simulink model "sparrow_albatros_spec_withgpio"  (R2021a)
settings: Solver=VariableStepDiscrete  StartTime=0.0  StopTime=100  RelTol=1e-3
undefined symbols (not defined in the file): pfb_coeff_gen_calc
libraries: xbsIndex_r4 x5582, casper_library_misc x33, casper_library_delays x28, xps_library x10, simulink x8, xbsReplacements_r4 x2
(part 8 of 80)

== system sparrow_albatros_spec_withgpio/reorder ==
  sync : Inport
  en : Inport  Port=2
  din0 : Inport  Port=3
  delay_din0 : xbsIndex_r4/Delay  rst=off  infoeditControl=Selection of Reset will increase slice count due to use of real FFs and instead of SRLs  en=off  latency=3  reg_retiming=on  dbl_ovrd=off  block_type=delay
  delay_din_bram0 : casper_library_delays/delay_bram_en_plus  DelayLen=length(map)  bram_latency=bram_latency+fanout_latency
      settings: SourceProductName=CASPER DSP Blockset
  delay_valid : xbsIndex_r4/Delay  rst=off  infoeditControl=Selection of Reset will increase slice count due to use of real FFs and instead of SRLs  en=off  latency=3  reg_retiming=on  dbl_ovrd=off  block_type=delay
  delay_we0 : xbsIndex_r4/Delay  rst=off  infoeditControl=Selection of Reset will increase slice count due to use of real FFs and instead of SRLs  en=off  latency=3  reg_retiming=on  dbl_ovrd=off  block_type=delay
  delay_we1 : xbsIndex_r4/Delay  rst=off  infoeditControl=Selection of Reset will increase slice count due to use of real FFs and instead of SRLs  en=off  latency=3  reg_retiming=on  dbl_ovrd=off  block_type=delay
  delay_we2 : xbsIndex_r4/Delay  rst=off  infoeditControl=Selection of Reset will increase slice count due to use of real FFs and instead of SRLs  en=off  latency=3  reg_retiming=on  dbl_ovrd=off  block_type=delay
  or : xbsIndex_r4/Logical  logical_function=OR  inputs=2  en=off  latency=0  precision=Full  arith_type=Unsigned  n_bits=16  bin_pt=0  align_bp=on  dbl_ovrd=off  block_type=logical
  post_sync_delay : xbsIndex_r4/Delay  rst=off  infoeditControl=Selection of Reset will increase slice count due to use of real FFs and instead of SRLs  en=off  latency=3  reg_retiming=on  dbl_ovrd=off  block_type=delay
  pre_sync_delay : xbsIndex_r4/Delay  rst=off  infoeditControl=Selection of Reset will increase slice count due to use of real FFs and instead of SRLs  en=off  latency=3  reg_retiming=on  dbl_ovrd=off  block_type=delay
  sync_delay_en : casper_library_delays/sync_delay_en  DelayLen=2048
      settings: SourceProductName=CASPER DSP Blockset
  we_expand : Subsystem  AncestorBlock=casper_library_flow_control/bus_expand  mask(bus_expand){mode=divisions of equal size, outputNum=1, outputWidth=1, outputBinaryPt=0, outputArithmeticType=2, show_format=off, outputToWorkspace=off, variablePrefix=out, outputToModelAsWell=on}
      mask prompts: outputNum "Number of outputs:"; outputWidth "Output width:"; outputBinaryPt "Output binary point position:"; outputArithmeticType "Output arithmetic type (ufix=0, fix=1, bool=2):"; show_format "Print format string?"; outputToWorkspace "Output to workspace?"; variablePrefix "Variable name prefix:"; outputToModelAsWell "Output to model as well?"
      mask help:
      | Expands a 'bus' made using a bus_create or Xilinx
      | concat block.
      | The input will be divided into the specified number
      | of outputs with the specified arithmetic types.
      | Divisions are made from most significant bit.
      mask init: same as sparrow_albatros_spec_withgpio/bus_expand
      settings: AttributesFormatString=1 outputs
      mask TypeOptions mode: divisions of equal size | divisions of arbitrary size
      mask Callback mode: %bus_expand_callback();
      mask Callback outputWidth: %bus_expand_callback();
      mask Callback outputToWorkspace: %bus_expand_callback();
  we_replicate : Subsystem  AncestorBlock=casper_library_bus/bus_replicate  mask(bus_replicate){replication=1, csp_latency=0, misc=off, implementation=core}
      mask prompts: replication "replication factor"; csp_latency "latency"; misc "misc support"; implementation "delay implementation"
      mask help: Output bus formed by replicating input bus a number of times
      mask init:
      | bus_replicate_init(gcb, ...
      |     'replication', replication, ...
      |     'csp_latency', csp_latency, ...
      |     'implementation', implementation, ...
      |     'misc', misc);
      mask TypeOptions implementation: core | behavioral
  sync_out : Outport
  valid : Outport  Port=2
  dout0 : Outport  Port=3
  wires:
  en/1 -> delay_we0/1, delay_we1/1, delay_we2/1
  delay_we1/1 -> delay_valid/1
  delay_valid/1 -> valid/1
  delay_we2/1 -> we_replicate/1(in)
  we_replicate/1(out) -> we_expand/1(bus_in)
  sync/1 -> pre_sync_delay/1
  delay_we0/1 -> or/2
  pre_sync_delay/1 -> or/1, sync_delay_en/1
  or/1 -> sync_delay_en/2
  sync_delay_en/1 -> post_sync_delay/1
  post_sync_delay/1 -> sync_out/1
  din0/1 -> delay_din0/1
  delay_din0/1 -> delay_din_bram0/1
  delay_din_bram0/1 -> dout0/1
  we_expand/1(msb_lsb_out1) -> delay_din_bram0/2

== system sparrow_albatros_spec_withgpio/sel ==
  sim_1 : Inport
  convert1_1 : DataTypeConversion  OutDataTypeStr=fixdt('ufix1_En0')  LockScale=on
  convert2_1 : DataTypeConversion  OutDataTypeStr=fixdt('ufix1_En0')  ConvertRealWorld=Stored Integer (SI)  LockScale=on
  gain_1 : Gain  OutDataTypeStr=fixdt('ufix32_En0')
  io_delay : xbsIndex_r4/Delay  rst=off  infoeditControl=Selection of Reset will increase slice count due to use of real FFs and instead of SRLs  en=off  latency=0  reg_retiming=on  dbl_ovrd=off  block_type=delay
  slice_reg : xbsIndex_r4/Slice  nbits=1  boolean_output=on  mode=Lower Bit Location + Width  bit1=0  base1=MSB of Input  bit0=0  base0=LSB of Input  dbl_ovrd=off  block_type=slice
  sparrow_albatros_spec_withgpio_sel_user_data_out : xbsIndex_r4/Gateway In  gui_display_data_type=Fixed-point  arith_type=Unsigned  n_bits=32  bin_pt=0  preci_type=Single  exp_width=8  frac_width=24  rows=1  columns=1  quantization="Round  (unbiased: +/- Inf)"  overflow=Saturate  period=1  UseAsADC=off  ADCChannel='1'  interface=None  automatic_assignment=on  address_offset=hex2dec('00')  intf_name=''  intf_description=''  default_value=0  timing_constraint=None  locs_specified=off  LOCs={}  io_standard={}  inherit_from_input=off  hdl_port=on  dbl_ovrd=off  block_type=gatewayin
  in_reg : Outport  VectorParamsAs1DForOutWhenUnconnected=off
  wires:
  sparrow_albatros_spec_withgpio_sel_user_data_out/1 -> io_delay/1
  sim_1/1 -> convert1_1/1
  convert1_1/1 -> convert2_1/1
  convert2_1/1 -> gain_1/1
  gain_1/1 -> sparrow_albatros_spec_withgpio_sel_user_data_out/1
  io_delay/1 -> slice_reg/1
  slice_reg/1 -> in_reg/1

== system sparrow_albatros_spec_withgpio/sim_pulse_gen ==
  Compare To Constant : simulink/Logic and Bit Operations/Compare To Constant  relop===  const=delay  OutDataTypeStr=boolean
  Counter Limited : simulink/Sources/Counter Limited  uplimit=delay+1  tsamp=-1
  Logical Operator : Logic  AllPortsSameDT=off  OutDataTypeStr=boolean
  Logical Operator1 : Logic  AllPortsSameDT=off  OutDataTypeStr=boolean
  Logical Operator2 : Logic  Operator=NOT  AllPortsSameDT=off  OutDataTypeStr=boolean
  Memory : Memory  InitialCondition=1
  Out1 : Outport
  wires:
  Logical Operator1/1 -> Memory/1
  Logical Operator/1 -> Out1/1, Logical Operator2/1
  Counter Limited/1 -> Compare To Constant/1
  Compare To Constant/1 -> Logical Operator/1
  Logical Operator2/1 -> Logical Operator1/2
  Memory/1 -> Logical Operator1/1, Logical Operator/2

== system sparrow_albatros_spec_withgpio/sim_pulse_gen1 ==
  Compare To Constant : simulink/Logic and Bit Operations/Compare To Constant  relop===  const=delay  OutDataTypeStr=boolean
  Counter Limited : simulink/Sources/Counter Limited  uplimit=delay+1  tsamp=-1
  Logical Operator : Logic  AllPortsSameDT=off  OutDataTypeStr=boolean
  Logical Operator1 : Logic  AllPortsSameDT=off  OutDataTypeStr=boolean
  Logical Operator2 : Logic  Operator=NOT  AllPortsSameDT=off  OutDataTypeStr=boolean
  Memory : Memory  InitialCondition=1
  Out1 : Outport
  wires:
  Memory/1 -> Logical Operator/2, Logical Operator1/1
  Logical Operator2/1 -> Logical Operator1/2
  Compare To Constant/1 -> Logical Operator/1
  Counter Limited/1 -> Compare To Constant/1
  Logical Operator/1 -> Logical Operator2/1, Out1/1
  Logical Operator1/1 -> Memory/1

== system sparrow_albatros_spec_withgpio/sim_pulse_gen2 ==
  Compare To Constant : simulink/Logic and Bit Operations/Compare To Constant  relop===  const=delay  OutDataTypeStr=boolean
  Counter Limited : simulink/Sources/Counter Limited  uplimit=delay+1  tsamp=-1
  Logical Operator : Logic  AllPortsSameDT=off  OutDataTypeStr=boolean
  Logical Operator1 : Logic  AllPortsSameDT=off  OutDataTypeStr=boolean
  Logical Operator2 : Logic  Operator=NOT  AllPortsSameDT=off  OutDataTypeStr=boolean
  Memory : Memory  InitialCondition=1
  Out1 : Outport
  wires:
  Logical Operator1/1 -> Memory/1
  Logical Operator/1 -> Out1/1, Logical Operator2/1
  Counter Limited/1 -> Compare To Constant/1
  Compare To Constant/1 -> Logical Operator/1
  Logical Operator2/1 -> Logical Operator1/2
  Memory/1 -> Logical Operator1/1, Logical Operator/2

== system sparrow_albatros_spec_withgpio/simple_bram_vacc2 ==
  new_acc : Inport
  din : Inport  Port=2
  Adder : xbsIndex_r4/AddSub  mode=Addition  use_carryin=off  use_carryout=off  en=off  latency=2  precision=User Defined  arith_type=Unsigned  n_bits=n_bits  bin_pt=bin_pt  quantization=Truncate  overflow=Wrap  use_behavioral_HDL=on  hw_selection=Fabric  pipelined=off  use_rpm=on  dbl_ovrd=off  block_type=addsub
      settings: xl_area=[0, 0, 0, 0, 0, 0, 0]  block_version=10.1.3
  Constant : xbsIndex_r4/Constant  const=0  gui_display_data_type=Fixed-point  arith_type=Unsigned  n_bits=n_bits  bin_pt=bin_pt  preci_type=Single  exp_width=8  frac_width=24  explicit_period=on  period=1  equ=P=C  opselect=C  inp2=PCIN>>17  opr=+  inp1=P  carry=CIN  dbl_ovrd=off  block_type=constant
  Mux : xbsIndex_r4/Mux  inputs=2  en=off  latency=0  precision=Full  arith_type="Signed  (2's comp)"  n_bits=8  bin_pt=2  quantization=Truncate  overflow=Wrap  dbl_ovrd=off  block_type=mux
      settings: xl_area=[0, 0, 0, 0, 0, 0, 0]
  delay_bram : Subsystem  mask(delay_bram){DelayLen=vec_len - 2, bram_latency=2}
      mask prompts: DelayLen "Delay By:"; bram_latency "BRAM Latency"
      mask help: A delay block that uses BRAM for its storage.
      mask init:
      | if (DelayLen <= bram_latency)
      | 	error('delay value must be greater than BRAM Latency');
      | end
      | BitWidth = max(ceil(log2(DelayLen)), 2);
      mask Help: eval('xlWeb(''http://casper.berkeley.edu/wiki/Delay_bram'')')
  pulse_ext : Subsystem  mask(pulse_ext){pulse_len=vec_len}
      mask prompts: pulse_len "Length of Pulse"
      mask help:
      | Extends a boolean signal to be high for the specified number of clocks after
      | the last high input.
      mask init:
      | bits = ceil(log2(pulse_len+1));
      mask Help: eval('xlWeb(''http://casper.berkeley.edu/wiki/Pulse_ext'')')
  dout : Outport  VectorParamsAs1DForOutWhenUnconnected=off
  valid : Outport  Port=2  VectorParamsAs1DForOutWhenUnconnected=off
  wires:
  Adder/1 -> delay_bram/1(In1)
  delay_bram/1(Out1) -> dout/1, Mux/2
  new_acc/1 -> pulse_ext/1(in)
  din/1 -> Adder/1
  pulse_ext/1(out) -> valid/1, Mux/1
  Mux/1 -> Adder/2
  Constant/1 -> Mux/3

== system sparrow_albatros_spec_withgpio/simple_bram_vacc3 ==
  new_acc : Inport
  din : Inport  Port=2
  Adder : xbsIndex_r4/AddSub  mode=Addition  use_carryin=off  use_carryout=off  en=off  latency=2  precision=User Defined  arith_type=Unsigned  n_bits=n_bits  bin_pt=bin_pt  quantization=Truncate  overflow=Wrap  use_behavioral_HDL=on  hw_selection=Fabric  pipelined=off  use_rpm=on  dbl_ovrd=off  block_type=addsub
      settings: xl_area=[0, 0, 0, 0, 0, 0, 0]  block_version=10.1.3
  Constant : xbsIndex_r4/Constant  const=0  gui_display_data_type=Fixed-point  arith_type=Unsigned  n_bits=n_bits  bin_pt=bin_pt  preci_type=Single  exp_width=8  frac_width=24  explicit_period=on  period=1  equ=P=C  opselect=C  inp2=PCIN>>17  opr=+  inp1=P  carry=CIN  dbl_ovrd=off  block_type=constant
  Mux : xbsIndex_r4/Mux  inputs=2  en=off  latency=0  precision=Full  arith_type="Signed  (2's comp)"  n_bits=8  bin_pt=2  quantization=Truncate  overflow=Wrap  dbl_ovrd=off  block_type=mux
      settings: xl_area=[0, 0, 0, 0, 0, 0, 0]
  delay_bram : Subsystem  mask(delay_bram){DelayLen=vec_len - 2, bram_latency=2}
      mask prompts: DelayLen "Delay By:"; bram_latency "BRAM Latency"
      mask help: A delay block that uses BRAM for its storage.
      mask init:
      | if (DelayLen <= bram_latency)
      | 	error('delay value must be greater than BRAM Latency');
      | end
      | BitWidth = max(ceil(log2(DelayLen)), 2);
      mask Help: eval('xlWeb(''http://casper.berkeley.edu/wiki/Delay_bram'')')
  pulse_ext : Subsystem  mask(pulse_ext){pulse_len=vec_len}
      mask prompts: pulse_len "Length of Pulse"
      mask help:
      | Extends a boolean signal to be high for the specified number of clocks after
      | the last high input.
      mask init:
      | bits = ceil(log2(pulse_len+1));
      mask Help: eval('xlWeb(''http://casper.berkeley.edu/wiki/Pulse_ext'')')
  dout : Outport  VectorParamsAs1DForOutWhenUnconnected=off
  valid : Outport  Port=2  VectorParamsAs1DForOutWhenUnconnected=off
  wires:
  Constant/1 -> Mux/3
  Mux/1 -> Adder/2
  pulse_ext/1(out) -> Mux/1, valid/1
  din/1 -> Adder/1
  new_acc/1 -> pulse_ext/1(in)
  delay_bram/1(Out1) -> Mux/2, dout/1
  Adder/1 -> delay_bram/1(In1)

== system sparrow_albatros_spec_withgpio/simple_bram_vacc4 ==
  new_acc : Inport
  din : Inport  Port=2
  Adder : xbsIndex_r4/AddSub  mode=Addition  use_carryin=off  use_carryout=off  en=off  latency=2  precision=User Defined  arith_type="Signed  (2's comp)"  n_bits=n_bits  bin_pt=bin_pt  quantization=Truncate  overflow=Wrap  use_behavioral_HDL=on  hw_selection=Fabric  pipelined=off  use_rpm=on  dbl_ovrd=off  block_type=addsub
      settings: xl_area=[0, 0, 0, 0, 0, 0, 0]  block_version=10.1.3
  Constant : xbsIndex_r4/Constant  const=0  gui_display_data_type=Fixed-point  arith_type=Signed (2's comp)  n_bits=n_bits  bin_pt=bin_pt  preci_type=Single  exp_width=8  frac_width=24  explicit_period=on  period=1  equ=P=C  opselect=C  inp2=PCIN>>17  opr=+  inp1=P  carry=CIN  dbl_ovrd=off  block_type=constant
  Mux : xbsIndex_r4/Mux  inputs=2  en=off  latency=0  precision=Full  arith_type="Signed  (2's comp)"  n_bits=8  bin_pt=2  quantization=Truncate  overflow=Wrap  dbl_ovrd=off  block_type=mux
      settings: xl_area=[0, 0, 0, 0, 0, 0, 0]
  delay_bram : Subsystem  mask(delay_bram){DelayLen=vec_len - 2, bram_latency=2}
      mask prompts: DelayLen "Delay By:"; bram_latency "BRAM Latency"
      mask help: A delay block that uses BRAM for its storage.
      mask init:
      | if (DelayLen <= bram_latency)
      | 	error('delay value must be greater than BRAM Latency');
      | end
      | BitWidth = max(ceil(log2(DelayLen)), 2);
      mask Help: eval('xlWeb(''http://casper.berkeley.edu/wiki/Delay_bram'')')
  pulse_ext : Subsystem  mask(pulse_ext){pulse_len=vec_len}
      mask prompts: pulse_len "Length of Pulse"
      mask help:
      | Extends a boolean signal to be high for the specified number of clocks after
      | the last high input.
      mask init:
      | bits = ceil(log2(pulse_len+1));
      mask Help: eval('xlWeb(''http://casper.berkeley.edu/wiki/Pulse_ext'')')
  dout : Outport  VectorParamsAs1DForOutWhenUnconnected=off
  valid : Outport  Port=2  VectorParamsAs1DForOutWhenUnconnected=off
  wires:
  Constant/1 -> Mux/3
  Mux/1 -> Adder/2
  pulse_ext/1(out) -> Mux/1, valid/1
  din/1 -> Adder/1
  new_acc/1 -> pulse_ext/1(in)
  delay_bram/1(Out1) -> Mux/2, dout/1
  Adder/1 -> delay_bram/1(In1)

== system sparrow_albatros_spec_withgpio/simple_bram_vacc5 ==
  new_acc : Inport
  din : Inport  Port=2
  Adder : xbsIndex_r4/AddSub  mode=Addition  use_carryin=off  use_carryout=off  en=off  latency=2  precision=User Defined  arith_type="Signed  (2's comp)"  n_bits=n_bits  bin_pt=bin_pt  quantization=Truncate  overflow=Wrap  use_behavioral_HDL=on  hw_selection=Fabric  pipelined=off  use_rpm=on  dbl_ovrd=off  block_type=addsub
      settings: xl_area=[0, 0, 0, 0, 0, 0, 0]  block_version=10.1.3
  Constant : xbsIndex_r4/Constant  const=0  gui_display_data_type=Fixed-point  arith_type=Signed (2's comp)  n_bits=n_bits  bin_pt=bin_pt  preci_type=Single  exp_width=8  frac_width=24  explicit_period=on  period=1  equ=P=C  opselect=C  inp2=PCIN>>17  opr=+  inp1=P  carry=CIN  dbl_ovrd=off  block_type=constant
  Mux : xbsIndex_r4/Mux  inputs=2  en=off  latency=0  precision=Full  arith_type="Signed  (2's comp)"  n_bits=8  bin_pt=2  quantization=Truncate  overflow=Wrap  dbl_ovrd=off  block_type=mux
      settings: xl_area=[0, 0, 0, 0, 0, 0, 0]
  delay_bram : Subsystem  mask(delay_bram){DelayLen=vec_len - 2, bram_latency=2}
      mask prompts: DelayLen "Delay By:"; bram_latency "BRAM Latency"
      mask help: A delay block that uses BRAM for its storage.
      mask init:
      | if (DelayLen <= bram_latency)
      | 	error('delay value must be greater than BRAM Latency');
      | end
      | BitWidth = max(ceil(log2(DelayLen)), 2);
      mask Help: eval('xlWeb(''http://casper.berkeley.edu/wiki/Delay_bram'')')
  pulse_ext : Subsystem  mask(pulse_ext){pulse_len=vec_len}
      mask prompts: pulse_len "Length of Pulse"
      mask help:
      | Extends a boolean signal to be high for the specified number of clocks after
      | the last high input.
      mask init:
      | bits = ceil(log2(pulse_len+1));
      mask Help: eval('xlWeb(''http://casper.berkeley.edu/wiki/Pulse_ext'')')
  dout : Outport  VectorParamsAs1DForOutWhenUnconnected=off
  valid : Outport  Port=2  VectorParamsAs1DForOutWhenUnconnected=off
  wires:
  Adder/1 -> delay_bram/1(In1)
  delay_bram/1(Out1) -> dout/1, Mux/2
  new_acc/1 -> pulse_ext/1(in)
  din/1 -> Adder/1
  pulse_ext/1(out) -> valid/1, Mux/1
  Mux/1 -> Adder/2
  Constant/1 -> Mux/3

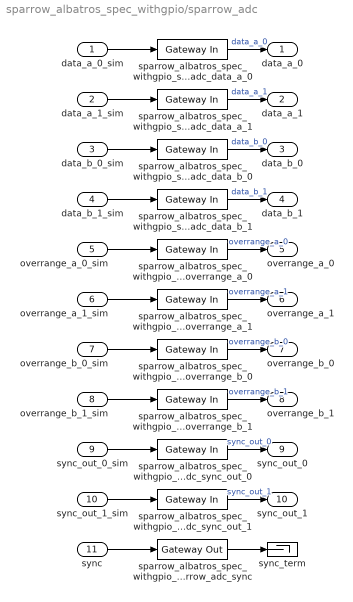
== system sparrow_albatros_spec_withgpio/sparrow_adc ==
  data_a_0_sim : Inport
  data_a_1_sim : Inport  Port=2
  data_b_0_sim : Inport  Port=3
  data_b_1_sim : Inport  Port=4
  overrange_a_0_sim : Inport  Port=5
  overrange_a_1_sim : Inport  Port=6
  overrange_b_0_sim : Inport  Port=7
  overrange_b_1_sim : Inport  Port=8
  sync_out_0_sim : Inport  Port=9
  sync_out_1_sim : Inport  Port=10
  sync : Inport  Port=11
  sparrow_albatros_spec_withgpio_sparrow_adc_data_a_0 : xbsIndex_r4/Gateway In  gui_display_data_type=Fixed-point  arith_type="Signed  (2's comp)"  n_bits=12  bin_pt=11  preci_type=Single  exp_width=8  frac_width=24  rows=1  columns=1  quantization="Round  (unbiased: +/- Inf)"  overflow=Saturate  period=1  UseAsADC=off  ADCChannel='1'  interface=None  automatic_assignment=on  address_offset=hex2dec('00')  intf_name=''  intf_description=''  default_value=0  timing_constraint=None  locs_specified=off  LOCs={}  io_standard={}  inherit_from_input=off  hdl_port=on  dbl_ovrd=off  block_type=gatewayin
  sparrow_albatros_spec_withgpio_sparrow_adc_data_a_1 : xbsIndex_r4/Gateway In  gui_display_data_type=Fixed-point  arith_type="Signed  (2's comp)"  n_bits=12  bin_pt=11  preci_type=Single  exp_width=8  frac_width=24  rows=1  columns=1  quantization="Round  (unbiased: +/- Inf)"  overflow=Saturate  period=1  UseAsADC=off  ADCChannel='1'  interface=None  automatic_assignment=on  address_offset=hex2dec('00')  intf_name=''  intf_description=''  default_value=0  timing_constraint=None  locs_specified=off  LOCs={}  io_standard={}  inherit_from_input=off  hdl_port=on  dbl_ovrd=off  block_type=gatewayin
  sparrow_albatros_spec_withgpio_sparrow_adc_data_b_0 : xbsIndex_r4/Gateway In  gui_display_data_type=Fixed-point  arith_type="Signed  (2's comp)"  n_bits=12  bin_pt=11  preci_type=Single  exp_width=8  frac_width=24  rows=1  columns=1  quantization="Round  (unbiased: +/- Inf)"  overflow=Saturate  period=1  UseAsADC=off  ADCChannel='1'  interface=None  automatic_assignment=on  address_offset=hex2dec('00')  intf_name=''  intf_description=''  default_value=0  timing_constraint=None  locs_specified=off  LOCs={}  io_standard={}  inherit_from_input=off  hdl_port=on  dbl_ovrd=off  block_type=gatewayin
  sparrow_albatros_spec_withgpio_sparrow_adc_data_b_1 : xbsIndex_r4/Gateway In  gui_display_data_type=Fixed-point  arith_type="Signed  (2's comp)"  n_bits=12  bin_pt=11  preci_type=Single  exp_width=8  frac_width=24  rows=1  columns=1  quantization="Round  (unbiased: +/- Inf)"  overflow=Saturate  period=1  UseAsADC=off  ADCChannel='1'  interface=None  automatic_assignment=on  address_offset=hex2dec('00')  intf_name=''  intf_description=''  default_value=0  timing_constraint=None  locs_specified=off  LOCs={}  io_standard={}  inherit_from_input=off  hdl_port=on  dbl_ovrd=off  block_type=gatewayin
  sparrow_albatros_spec_withgpio_sparrow_adc_overrange_a_0 : xbsIndex_r4/Gateway In  gui_display_data_type=Fixed-point  arith_type=Boolean  n_bits=1  bin_pt=0  preci_type=Single  exp_width=8  frac_width=24  rows=1  columns=1  quantization="Round  (unbiased: +/- Inf)"  overflow=Saturate  period=1  UseAsADC=off  ADCChannel='1'  interface=None  automatic_assignment=on  address_offset=hex2dec('00')  intf_name=''  intf_description=''  default_value=0  timing_constraint=None  locs_specified=off  LOCs={}  io_standard={}  inherit_from_input=off  hdl_port=on  dbl_ovrd=off  block_type=gatewayin
  sparrow_albatros_spec_withgpio_sparrow_adc_overrange_a_1 : xbsIndex_r4/Gateway In  gui_display_data_type=Fixed-point  arith_type=Boolean  n_bits=1  bin_pt=0  preci_type=Single  exp_width=8  frac_width=24  rows=1  columns=1  quantization="Round  (unbiased: +/- Inf)"  overflow=Saturate  period=1  UseAsADC=off  ADCChannel='1'  interface=None  automatic_assignment=on  address_offset=hex2dec('00')  intf_name=''  intf_description=''  default_value=0  timing_constraint=None  locs_specified=off  LOCs={}  io_standard={}  inherit_from_input=off  hdl_port=on  dbl_ovrd=off  block_type=gatewayin
  sparrow_albatros_spec_withgpio_sparrow_adc_overrange_b_0 : xbsIndex_r4/Gateway In  gui_display_data_type=Fixed-point  arith_type=Boolean  n_bits=1  bin_pt=0  preci_type=Single  exp_width=8  frac_width=24  rows=1  columns=1  quantization="Round  (unbiased: +/- Inf)"  overflow=Saturate  period=1  UseAsADC=off  ADCChannel='1'  interface=None  automatic_assignment=on  address_offset=hex2dec('00')  intf_name=''  intf_description=''  default_value=0  timing_constraint=None  locs_specified=off  LOCs={}  io_standard={}  inherit_from_input=off  hdl_port=on  dbl_ovrd=off  block_type=gatewayin
  sparrow_albatros_spec_withgpio_sparrow_adc_overrange_b_1 : xbsIndex_r4/Gateway In  gui_display_data_type=Fixed-point  arith_type=Boolean  n_bits=1  bin_pt=0  preci_type=Single  exp_width=8  frac_width=24  rows=1  columns=1  quantization="Round  (unbiased: +/- Inf)"  overflow=Saturate  period=1  UseAsADC=off  ADCChannel='1'  interface=None  automatic_assignment=on  address_offset=hex2dec('00')  intf_name=''  intf_description=''  default_value=0  timing_constraint=None  locs_specified=off  LOCs={}  io_standard={}  inherit_from_input=off  hdl_port=on  dbl_ovrd=off  block_type=gatewayin
  sparrow_albatros_spec_withgpio_sparrow_adc_sync : xbsIndex_r4/Gateway Out  inherit_from_input=off  hdl_port=on  rows=1  columns=1  UseAsDAC=off  DACChannel='1'  interface=None  automatic_assignment=on  address_offset=hex2dec('00')  intf_name=''  intf_description=''  timing_constraint=None  locs_specified=off  LOCs={}  io_standard={}  block_type=gatewayout
  sparrow_albatros_spec_withgpio_sparrow_adc_sync_out_0 : xbsIndex_r4/Gateway In  gui_display_data_type=Fixed-point  arith_type=Boolean  n_bits=1  bin_pt=0  preci_type=Single  exp_width=8  frac_width=24  rows=1  columns=1  quantization="Round  (unbiased: +/- Inf)"  overflow=Saturate  period=1  UseAsADC=off  ADCChannel='1'  interface=None  automatic_assignment=on  address_offset=hex2dec('00')  intf_name=''  intf_description=''  default_value=0  timing_constraint=None  locs_specified=off  LOCs={}  io_standard={}  inherit_from_input=off  hdl_port=on  dbl_ovrd=off  block_type=gatewayin
  sparrow_albatros_spec_withgpio_sparrow_adc_sync_out_1 : xbsIndex_r4/Gateway In  gui_display_data_type=Fixed-point  arith_type=Boolean  n_bits=1  bin_pt=0  preci_type=Single  exp_width=8  frac_width=24  rows=1  columns=1  quantization="Round  (unbiased: +/- Inf)"  overflow=Saturate  period=1  UseAsADC=off  ADCChannel='1'  interface=None  automatic_assignment=on  address_offset=hex2dec('00')  intf_name=''  intf_description=''  default_value=0  timing_constraint=None  locs_specified=off  LOCs={}  io_standard={}  inherit_from_input=off  hdl_port=on  dbl_ovrd=off  block_type=gatewayin
  sync_term : Terminator
  data_a_0 : Outport  VectorParamsAs1DForOutWhenUnconnected=off
  data_a_1 : Outport  Port=2  VectorParamsAs1DForOutWhenUnconnected=off
  data_b_0 : Outport  Port=3  VectorParamsAs1DForOutWhenUnconnected=off
  data_b_1 : Outport  Port=4  VectorParamsAs1DForOutWhenUnconnected=off
  overrange_a_0 : Outport  Port=5  VectorParamsAs1DForOutWhenUnconnected=off
  overrange_a_1 : Outport  Port=6  VectorParamsAs1DForOutWhenUnconnected=off
  overrange_b_0 : Outport  Port=7  VectorParamsAs1DForOutWhenUnconnected=off
  overrange_b_1 : Outport  Port=8  VectorParamsAs1DForOutWhenUnconnected=off
  sync_out_0 : Outport  Port=9  VectorParamsAs1DForOutWhenUnconnected=off
  sync_out_1 : Outport  Port=10  VectorParamsAs1DForOutWhenUnconnected=off
  wires:
  data_a_0_sim/1 -> sparrow_albatros_spec_withgpio_sparrow_adc_data_a_0/1
  sparrow_albatros_spec_withgpio_sparrow_adc_data_a_0/1 -> data_a_0/1  "data_a_0"
  data_a_1_sim/1 -> sparrow_albatros_spec_withgpio_sparrow_adc_data_a_1/1
  sparrow_albatros_spec_withgpio_sparrow_adc_data_a_1/1 -> data_a_1/1  "data_a_1"
  data_b_0_sim/1 -> sparrow_albatros_spec_withgpio_sparrow_adc_data_b_0/1
  sparrow_albatros_spec_withgpio_sparrow_adc_data_b_0/1 -> data_b_0/1  "data_b_0"
  data_b_1_sim/1 -> sparrow_albatros_spec_withgpio_sparrow_adc_data_b_1/1
  sparrow_albatros_spec_withgpio_sparrow_adc_data_b_1/1 -> data_b_1/1  "data_b_1"
  overrange_a_0_sim/1 -> sparrow_albatros_spec_withgpio_sparrow_adc_overrange_a_0/1
  sparrow_albatros_spec_withgpio_sparrow_adc_overrange_a_0/1 -> overrange_a_0/1  "overrange_a_0"
  overrange_a_1_sim/1 -> sparrow_albatros_spec_withgpio_sparrow_adc_overrange_a_1/1
  sparrow_albatros_spec_withgpio_sparrow_adc_overrange_a_1/1 -> overrange_a_1/1  "overrange_a_1"
  overrange_b_0_sim/1 -> sparrow_albatros_spec_withgpio_sparrow_adc_overrange_b_0/1
  sparrow_albatros_spec_withgpio_sparrow_adc_overrange_b_0/1 -> overrange_b_0/1  "overrange_b_0"
  overrange_b_1_sim/1 -> sparrow_albatros_spec_withgpio_sparrow_adc_overrange_b_1/1
  sparrow_albatros_spec_withgpio_sparrow_adc_overrange_b_1/1 -> overrange_b_1/1  "overrange_b_1"
  sync_out_0_sim/1 -> sparrow_albatros_spec_withgpio_sparrow_adc_sync_out_0/1
  sparrow_albatros_spec_withgpio_sparrow_adc_sync_out_0/1 -> sync_out_0/1  "sync_out_0"
  sync_out_1_sim/1 -> sparrow_albatros_spec_withgpio_sparrow_adc_sync_out_1/1
  sparrow_albatros_spec_withgpio_sparrow_adc_sync_out_1/1 -> sync_out_1/1  "sync_out_1"
  sync/1 -> sparrow_albatros_spec_withgpio_sparrow_adc_sync/1
  sparrow_albatros_spec_withgpio_sparrow_adc_sync/1 -> sync_term/1

== system sparrow_albatros_spec_withgpio/square_transposer ==
  sync : Inport
  in0 : Inport  Port=2
  in1 : Inport  Port=3
  barrel_switcher : Subsystem  AncestorBlock=casper_library_reorder/barrel_switcher  mask(barrel_switcher){n_inputs=1, async=off}
      mask prompts: n_inputs "Number of Inputs: (2^?)"; async "Asynchronous operation"
      mask help:
      | Shifts input to right by amount specified on sel,
      | wrapping around into higher order bits.
      mask init:
      | barrel_switcher_init(gcb,...
      |     'n_inputs', n_inputs, ...
      |     'async', async);
      mask Help: eval('xlWeb(''http://casper.berkeley.edu/wiki/Barrel_switcher'')')
  counter : xbsIndex_r4/Counter  cnt_type=Free Running  cnt_to=Inf  operation=Down  start_count=0  cnt_by_val=1  arith_type=Unsigned  n_bits=n_inputs  bin_pt=0  load_pin=off  rst=on  en=off  explicit_period=on  period=1  use_behavioral_HDL=off  implementation=Fabric  dbl_ovrd=off  block_type=counter
  db0 : Subsystem  AncestorBlock=casper_library_delays/delay_slr  mask(delay_slr){DelayLen=1, async=off}
      mask prompts: DelayLen "Delay by:"; async "asynchronous operation"
      mask help: A delay block that uses slices (SLR16s) for its storage.
      mask init:
      | delay_slr_init(gcb, ...
      |     'DelayLen', DelayLen, ...
      |     'async', async);
  df1 : Subsystem  AncestorBlock=casper_library_delays/delay_slr  mask(delay_slr){DelayLen=1, async=off}
      mask prompts: DelayLen "Delay by:"; async "asynchronous operation"
      mask help: A delay block that uses slices (SLR16s) for its storage.
      mask init:
      | delay_slr_init(gcb, ...
      |     'DelayLen', DelayLen, ...
      |     'async', async);
  dsync : Subsystem  AncestorBlock=casper_library_delays/delay_slr  mask(delay_slr){DelayLen=1, async=off}
      mask prompts: DelayLen "Delay by:"; async "asynchronous operation"
      mask help: A delay block that uses slices (SLR16s) for its storage.
      mask init:
      | delay_slr_init(gcb, ...
      |     'DelayLen', DelayLen, ...
      |     'async', async);
  sync_out : Outport  VectorParamsAs1DForOutWhenUnconnected=off
  out0 : Outport  Port=2  VectorParamsAs1DForOutWhenUnconnected=off
  out1 : Outport  Port=3  VectorParamsAs1DForOutWhenUnconnected=off
  wires:
  sync/1 -> counter/1, barrel_switcher/2(sync_in)
  dsync/1(dout) -> sync_out/1
  counter/1 -> barrel_switcher/1(sel)
  barrel_switcher/1(sync_out) -> dsync/1(din)
  in0/1 -> barrel_switcher/3(In1)
  barrel_switcher/2(Out1) -> db0/1(din)
  db0/1(dout) -> out0/1
  in1/1 -> df1/1(din)
  df1/1(dout) -> barrel_switcher/4(In2)
  barrel_switcher/3(Out2) -> out1/1

== system sparrow_albatros_spec_withgpio/ss_adc ==
  note: Value on vin
      | aligned with
      | first sample on
      | din captured
  note: Number of valid
      | data samples to
      | skip after trigger
      | before starting
      | capture
  note: Number of
      | bytes in
      | buffer and
      | done bit
  note: Offset in vector
      | from first element
      | captured, used
      | during circular capture
  note: ctrl:
      | bit0: Put a posedge here
      |         to enable a new capture.
      | bit1: ignore external trigger
      |         and trigger immediately.
      | bit2: ignore external write
      |         enable and capture on
      |         every FPGA clock.
      | bit3: continuously capture
      |         data until we get an
      |         external stop command.
  note: Delay start
      | of capture
  note: Generate stop
      | when in circular
      | capture mode
  din : Inport
  we : Inport  Port=2
  trig : Inport  Port=3
  add_del : xbsIndex_r4/Delay  rst=off  infoeditControl=Selection of Reset will increase slice count due to use of real FFs and instead of SRLs  en=off  latency=1  reg_retiming=on  dbl_ovrd=off  block_type=delay
      settings: block_version=11.4
  add_gen : Subsystem  AncestorBlock=casper_library_scopes/snapshot/add_gen  mask{counter_size=11+3+1, increment=8, nsamples=11, burst_size=0, use_dsp48=off}
      mask prompts: counter_size "Address counter size (2^?)"; increment "Address counter increment"; nsamples "Number of samples (2^?)"; burst_size "Burst size (2^?)"; use_dsp48 "dsp48 counter/s"
      mask init:
      | set_param(gcb,'LinkStatus','inactive');
      | if strcmp(use_dsp48,'on'),
      |     set_param([gcb,'/add_gen'],'implementation','DSP48');
      | else
      |     set_param([gcb,'/add_gen'],'implementation','Fabric');
      | end
  arm : xbsIndex_r4/Constant  const=0  gui_display_data_type=Fixed-point  arith_type=Boolean  n_bits=16  bin_pt=14  preci_type=Single  exp_width=8  frac_width=24  explicit_period=on  period=1  equ=P=C  opselect=C  inp2=PCIN>>17  opr=+  inp1=P  carry=CIN  dbl_ovrd=off  block_type=constant
  arm_or : xbsIndex_r4/Logical  logical_function=OR  inputs=2  en=off  latency=0  precision=Full  arith_type=Unsigned  n_bits=16  bin_pt=0  align_bp=on  dbl_ovrd=off  block_type=logical
  basic_ctrl : Subsystem  AncestorBlock=casper_library_scopes/snapshot/basic_ctrl  mask{dram=off, data_width=64}
      mask prompts: data_width "data width"
      mask init:
      | set_param(gcb,'LinkStatus','inactive');
      | set_param([gcb,'/dram_munge'], 'dram', dram);
  bram : Subsystem  Tag=xps:bram  AncestorBlock=xps_library/Memory/shared_bram  mask{arith_type=Unsigned, addr_width=11, data_width=64, reg_prim_output=off, reg_core_output=off, optimization=Minimum_Area, data_bin_pt=0, init_vals=[0:2^11-1], sample_rate=1}
      mask prompts: arith_type "Output Data Type"; addr_width "Address width"; data_width "Data Width"; reg_prim_output "Register Primitive Output"; reg_core_output "Register Core Output"; data_bin_pt "Data Binary Point"; init_vals "Initial values (simulation only)"; sample_rate "Sample rate"
      mask init:
      | shared_bram_mask;
      mask TypeOptions arith_type: Unsigned | Signed  (2's comp)
      mask TypeOptions data_width: 8 | 16 | 32 | 64 | 128
      mask TypeOptions optimization: Minimum_Area | Low_Power
  cast : xbsIndex_r4/Convert  gui_display_data_type=Fixed-point  arith_type=Unsigned  n_bits=64  bin_pt=0  float_type=Single  exp_bits=8  fraction_bits=24  quantization=Truncate  overflow=Wrap  en=off  latency=0  pipeline=off  dbl_ovrd=off  block_type=convert
      settings: block_version=11.4
  circ : xbsIndex_r4/Constant  const=0  gui_display_data_type=Fixed-point  arith_type=Boolean  n_bits=16  bin_pt=14  preci_type=Single  exp_width=8  frac_width=24  explicit_period=on  period=1  equ=P=C  opselect=C  inp2=PCIN>>17  opr=+  inp1=P  carry=CIN  dbl_ovrd=off  block_type=constant
  circ_or : xbsIndex_r4/Logical  logical_function=OR  inputs=2  en=off  latency=0  precision=Full  arith_type=Unsigned  n_bits=16  bin_pt=0  align_bp=on  dbl_ovrd=off  block_type=logical
  ctrl : Subsystem  Tag=xps:sw_reg  AncestorBlock=xps_library/Memory/software_register  mask(swreg){io_dir=From Processor, io_delay=0, init_val=0, sample_period=1, names=reg, bitwidths=32, bin_pts=0, arith_types=0, sim_port=off, show_format=on, desc_str=""}
      mask prompts: io_dir "I/O direction"; io_delay "I/O delay"; init_val "Initial Value"; sample_period "Sample period"; names "Bitfield names [msb...lsb]"; bitwidths "Bitfield widths"; bin_pts "Bitfield binary pts"; arith_types "Bitfield types, ufix=0, fix=1, bool=2"; sim_port "Provide sim input/output?"; show_format "Print format string?"; desc_str "Description"
      mask help: A 32-bit software-accessible register. Can be divided into bitfields of varying widths and types using the fields in the block mask.
      mask init:
      | swreg_init(gcb)
      settings: AttributesFormatString=1input:uf32.0 = 32 bits
      mask TypeOptions io_dir: To Processor | From Processor
      mask Callback io_dir:
      | mask_enables = get_param(gcb, 'MaskEnables');
      | mask_names = get_param(gcb, 'MaskNames');
      | if strcmp(get_param(gcb, 'io_dir'), 'To Processor'),
      |     mask_enables{ismember(mask_names, 'sample_period')} = 'off';
      | else
      |     mask_enables{ismember(mask_names, 'sample_period')} = 'on';
      | end
      | set_param(gcb, 'MaskEnables', mask_enables);
      mask DialogControl ParameterTabVar0 Prompt: Setup
  ctrl_combine : Subsystem  AncestorBlock=casper_library_flow_control/bus_create  mask(bus_create){inputNum=4}
      mask prompts: inputNum "Number of inputs:"
      mask init:
      | bus_create_init(gcb,...
      |     'inputNum', inputNum);
  ctrl_split : Subsystem  AncestorBlock=casper_library_flow_control/bus_expand  mask(bus_expand){mode=divisions of arbitrary size, outputNum=1, outputWidth=[28 1 2 1], outputBinaryPt=0, outputArithmeticType=[0 2 0 2], show_format=on, outputToWorkspace=off, variablePrefix=out, outputToModelAsWell=on}
      mask prompts: outputNum "Number of outputs:"; outputWidth "Output width [msb ... lsb]:"; outputBinaryPt "Output binary point position [msb ... lsb]:"; outputArithmeticType "Output arithmetic type (ufix=0, fix=1, bool=2) [msb ... lsb]:"; show_format "Print format string?"; outputToWorkspace "Output to workspace?"; variablePrefix "Variable name prefix:"; outputToModelAsWell "Output to model as well?"
      mask help:
      | Expands a 'bus' made using a bus_create or Xilinx
      | concat block.
      | The input will be divided into the specified number
      | of outputs with the specified arithmetic types.
      | Divisions are made from most significant bit.
      mask init: same as sparrow_albatros_spec_withgpio/bus_expand
      settings: AttributesFormatString=4 outputs: uf28.0,b,uf2.0,b,
      mask TypeOptions mode: divisions of equal size | divisions of arbitrary size
      mask Callback mode: bus_expand_callback();
      mask Callback outputWidth: bus_expand_callback();
      mask Callback outputToWorkspace: bus_expand_callback();
  dat_del : xbsIndex_r4/Delay  rst=off  infoeditControl=Selection of Reset will increase slice count due to use of real FFs and instead of SRLs  en=off  latency=1  reg_retiming=on  dbl_ovrd=off  block_type=delay
      settings: block_version=11.4
  g_tr_en_cnt : Terminator
  gbram : Terminator
  goto_ss_we2_const : xbsIndex_r4/Constant  const=0  gui_display_data_type=Fixed-point  arith_type=Boolean  n_bits=16  bin_pt=14  preci_type=Single  exp_width=8  frac_width=24  explicit_period=on  period=1  equ=P=C  opselect=C  inp2=PCIN>>17  opr=+  inp1=P  carry=CIN  dbl_ovrd=off  block_type=constant
  goto_ss_we3_const : xbsIndex_r4/Constant  const=0  gui_display_data_type=Fixed-point  arith_type=Boolean  n_bits=16  bin_pt=14  preci_type=Single  exp_width=8  frac_width=24  explicit_period=on  period=1  equ=P=C  opselect=C  inp2=PCIN>>17  opr=+  inp1=P  carry=CIN  dbl_ovrd=off  block_type=constant
  gval : Terminator
  never : xbsIndex_r4/Constant  const=0  gui_display_data_type=Fixed-point  arith_type=Boolean  n_bits=16  bin_pt=14  preci_type=Single  exp_width=8  frac_width=24  explicit_period=on  period=1  equ=P=C  opselect=C  inp2=PCIN>>17  opr=+  inp1=P  carry=CIN  dbl_ovrd=off  block_type=constant
  ri : xbsIndex_r4/Reinterpret  force_arith_type=on  arith_type=Unsigned  force_bin_pt=on  bin_pt=0  block_type=reinterpret
      settings: infoedit="Changes signal type without altering the binary representation.   You can changed the signal between signed and unsigned, and relocate the binary point.<br><br>Hardware notes: In hardware this block costs nothing.<br><br>Example:  Suppose the input is 6 bits wide, signed, with 2 fractional bits, and the output is forced to unsigned with 0 fractional bits.  Then an input of -2.0 (1110.00 in binary 2's complement) becomes an output of 56 (111000 in binary)."
  status : Subsystem  Tag=xps:sw_reg  AncestorBlock=xps_library/Memory/software_register  mask(swreg){io_dir=To Processor, io_delay=0, init_val=0, sample_period=1, names=reg, bitwidths=32, bin_pts=0, arith_types=0, sim_port=off, show_format=on, desc_str=""}
      mask prompts: io_dir "I/O direction"; io_delay "I/O delay"; init_val "Initial Value"; sample_period "Sample period"; names "Bitfield names [msb...lsb]"; bitwidths "Bitfield widths"; bin_pts "Bitfield binary pts"; arith_types "Bitfield types, ufix=0, fix=1, bool=2"; sim_port "Provide sim input/output?"; show_format "Print format string?"; desc_str "Description"
      mask help: A 32-bit software-accessible register. Can be divided into bitfields of varying widths and types using the fields in the block mask.
      mask init:
      | swreg_init(gcb)
      settings: AttributesFormatString=1output:uf32.0 = 32 bits
      mask TypeOptions io_dir: To Processor | From Processor
      mask Callback io_dir:
      | mask_enables = get_param(gcb, 'MaskEnables');
      | mask_names = get_param(gcb, 'MaskNames');
      | if strcmp(get_param(gcb, 'io_dir'), 'To Processor'),
      |     mask_enables{ismember(mask_names, 'sample_period')} = 'off';
      | else
      |     mask_enables{ismember(mask_names, 'sample_period')} = 'on';
      | end
      | set_param(gcb, 'MaskEnables', mask_enables);
      mask DialogControl ParameterTabVar0 Prompt: Setup
  vin_const : xbsIndex_r4/Constant  const=0  gui_display_data_type=Fixed-point  arith_type=Boolean  n_bits=16  bin_pt=14  preci_type=Single  exp_width=8  frac_width=24  explicit_period=on  period=1  equ=P=C  opselect=C  inp2=PCIN>>17  opr=+  inp1=P  carry=CIN  dbl_ovrd=off  block_type=constant
  we_del : xbsIndex_r4/Delay  rst=off  infoeditControl=Selection of Reset will increase slice count due to use of real FFs and instead of SRLs  en=off  latency=1  reg_retiming=on  dbl_ovrd=off  block_type=delay
      settings: block_version=11.4
  arm_out : Outport  VectorParamsAs1DForOutWhenUnconnected=off
  tag scope: goto_93113733_we1=global, goto_93113733_we2=global, goto_93113733_we3=global, goto_93113733_we4=global
  wires:
  din/1 -> ri/1
  ri/1 -> cast/1
  cast/1 -> basic_ctrl/2(din)
  we/1 -> basic_ctrl/3(we)
  trig/1 -> basic_ctrl/4(trig)
  ctrl_combine/1(bus_out) -> basic_ctrl/5(ctrl)
  never/1 -> basic_ctrl/6(stopi)
  arm/1 -> arm_or/2
  arm_or/1 -> arm_out/1, ctrl_combine/4(in4)
  circ/1 -> circ_or/2
  ctrl/1(in_reg) -> ctrl_split/1(bus_in)
  ctrl_split/1(msb_out4) -> ctrl_combine/1(in1)
  ctrl_split/2(out3) -> circ_or/1
  ctrl_split/3(out2) -> ctrl_combine/3(in3)
  ctrl_split/4(lsb_out1) -> arm_or/1
  circ_or/1 -> ctrl_combine/2(in2)
  basic_ctrl/1(vout) -> add_gen/1(vin)
  basic_ctrl/2(dout) -> add_gen/2(din)
  basic_ctrl/3(we_o) -> add_gen/3(we), [goto_93113733_we1]
  basic_ctrl/4(go) -> add_gen/4(go)
  basic_ctrl/5(stop) -> add_gen/5(cont)
  basic_ctrl/6(init) -> add_gen/6(init)
  add_gen/5(status) -> status/1(out_reg)
  vin_const/1 -> basic_ctrl/1(vin)
  add_gen/1(vout) -> gval/1
  add_gen/6(en_cnt) -> g_tr_en_cnt/1
  add_gen/2(add) -> add_del/1
  add_gen/3(dout) -> dat_del/1
  add_gen/4(we_o) -> we_del/1, [goto_93113733_we4]
  add_del/1 -> bram/1(addr)
  dat_del/1 -> bram/2(data_in)
  we_del/1 -> bram/3(we)
  bram/1(data_out) -> gbram/1
  goto_ss_we2_const/1 -> [goto_93113733_we2]
  goto_ss_we3_const/1 -> [goto_93113733_we3]

== system sparrow_albatros_spec_withgpio/sync ==
  sim_1 : Inport
  convert1_1 : DataTypeConversion  OutDataTypeStr=fixdt('ufix1_En0')  LockScale=on
  convert2_1 : DataTypeConversion  OutDataTypeStr=fixdt('ufix1_En0')  ConvertRealWorld=Stored Integer (SI)  LockScale=on
  gain_1 : Gain  OutDataTypeStr=fixdt('ufix32_En0')
  io_delay : xbsIndex_r4/Delay  rst=off  infoeditControl=Selection of Reset will increase slice count due to use of real FFs and instead of SRLs  en=off  latency=0  reg_retiming=on  dbl_ovrd=off  block_type=delay
  slice_reg : xbsIndex_r4/Slice  nbits=1  boolean_output=on  mode=Lower Bit Location + Width  bit1=0  base1=MSB of Input  bit0=0  base0=LSB of Input  dbl_ovrd=off  block_type=slice
  sparrow_albatros_spec_withgpio_sync_user_data_out : xbsIndex_r4/Gateway In  gui_display_data_type=Fixed-point  arith_type=Unsigned  n_bits=32  bin_pt=0  preci_type=Single  exp_width=8  frac_width=24  rows=1  columns=1  quantization="Round  (unbiased: +/- Inf)"  overflow=Saturate  period=1  UseAsADC=off  ADCChannel='1'  interface=None  automatic_assignment=on  address_offset=hex2dec('00')  intf_name=''  intf_description=''  default_value=0  timing_constraint=None  locs_specified=off  LOCs={}  io_standard={}  inherit_from_input=off  hdl_port=on  dbl_ovrd=off  block_type=gatewayin
  in_reg : Outport
  wires:
  sparrow_albatros_spec_withgpio_sync_user_data_out/1 -> io_delay/1
  sim_1/1 -> convert1_1/1
  convert1_1/1 -> convert2_1/1
  convert2_1/1 -> gain_1/1
  gain_1/1 -> sparrow_albatros_spec_withgpio_sync_user_data_out/1
  io_delay/1 -> slice_reg/1
  slice_reg/1 -> in_reg/1

== system sparrow_albatros_spec_withgpio/sync_adc ==
  sim_1 : Inport
  convert1_1 : DataTypeConversion  OutDataTypeStr=fixdt('ufix1_En0')  LockScale=on
  convert2_1 : DataTypeConversion  OutDataTypeStr=fixdt('ufix1_En0')  ConvertRealWorld=Stored Integer (SI)  LockScale=on
  gain_1 : Gain  OutDataTypeStr=fixdt('ufix32_En0')
  io_delay : xbsIndex_r4/Delay  rst=off  infoeditControl=Selection of Reset will increase slice count due to use of real FFs and instead of SRLs  en=off  latency=0  reg_retiming=on  dbl_ovrd=off  block_type=delay
  slice_reg : xbsIndex_r4/Slice  nbits=1  boolean_output=on  mode=Lower Bit Location + Width  bit1=0  base1=MSB of Input  bit0=0  base0=LSB of Input  dbl_ovrd=off  block_type=slice
  sparrow_albatros_spec_withgpio_sync_adc_user_data_out : xbsIndex_r4/Gateway In  gui_display_data_type=Fixed-point  arith_type=Unsigned  n_bits=32  bin_pt=0  preci_type=Single  exp_width=8  frac_width=24  rows=1  columns=1  quantization="Round  (unbiased: +/- Inf)"  overflow=Saturate  period=1  UseAsADC=off  ADCChannel='1'  interface=None  automatic_assignment=on  address_offset=hex2dec('00')  intf_name=''  intf_description=''  default_value=0  timing_constraint=None  locs_specified=off  LOCs={}  io_standard={}  inherit_from_input=off  hdl_port=on  dbl_ovrd=off  block_type=gatewayin
  in_reg : Outport
  wires:
  sparrow_albatros_spec_withgpio_sync_adc_user_data_out/1 -> io_delay/1
  sim_1/1 -> convert1_1/1
  convert1_1/1 -> convert2_1/1
  convert2_1/1 -> gain_1/1
  gain_1/1 -> sparrow_albatros_spec_withgpio_sync_adc_user_data_out/1
  io_delay/1 -> slice_reg/1
  slice_reg/1 -> in_reg/1

== system sparrow_albatros_spec_withgpio/sync_cnt ==
  out_reg : Inport
  assert_reg : xbsIndex_r4/Assert  assert_type=on  type_source=Explicitly  gui_display_data_type=Fixed-point  arith_type=Unsigned  n_bits=32  bin_pt=0  preci_type=Single  exp_width=8  frac_width=24  assert_rate=off  rate_source=Explicitly  period=1  output_port=on  block_type=assert
  cast_gw : xbsIndex_r4/Convert  gui_display_data_type=Fixed-point  arith_type=Unsigned  n_bits=32  bin_pt=0  float_type=Single  exp_bits=8  fraction_bits=24  quantization=Truncate  overflow=Wrap  en=off  latency=1  pipeline=off  dbl_ovrd=off  block_type=convert
  io_delay : xbsIndex_r4/Delay  rst=off  infoeditControl=Selection of Reset will increase slice count due to use of real FFs and instead of SRLs  en=off  latency=0  reg_retiming=on  dbl_ovrd=off  block_type=delay
  reint1 : xbsIndex_r4/Reinterpret  force_arith_type=on  arith_type=Unsigned  force_bin_pt=on  bin_pt=0  block_type=reinterpret
  sim_out : Terminator
  sim_out_reg_gw : xbsIndex_r4/Gateway Out  inherit_from_input=off  hdl_port=off  rows=1  columns=1  UseAsDAC=off  DACChannel='1'  interface=None  automatic_assignment=on  address_offset=hex2dec('00')  intf_name=''  intf_description=''  timing_constraint=None  locs_specified=off  LOCs={}  io_standard={}  block_type=gatewayout
  sim_out_reg_sim_delay : xbsIndex_r4/Delay  rst=off  infoeditControl=Selection of Reset will increase slice count due to use of real FFs and instead of SRLs  en=off  latency=1  reg_retiming=on  dbl_ovrd=off  block_type=delay
  sparrow_albatros_spec_withgpio_sync_cnt_user_data_in : xbsIndex_r4/Gateway Out  inherit_from_input=off  hdl_port=on  rows=1  columns=1  UseAsDAC=off  DACChannel='1'  interface=None  automatic_assignment=on  address_offset=hex2dec('00')  intf_name=''  intf_description=''  timing_constraint=None  locs_specified=off  LOCs={}  io_standard={}  block_type=gatewayout
  sim_out_reg : Outport  VectorParamsAs1DForOutWhenUnconnected=off
  wires:
  sim_out_reg_sim_delay/1 -> sim_out_reg_gw/1
  sim_out_reg_gw/1 -> sim_out_reg/1
  io_delay/1 -> cast_gw/1
  cast_gw/1 -> sparrow_albatros_spec_withgpio_sync_cnt_user_data_in/1
  sparrow_albatros_spec_withgpio_sync_cnt_user_data_in/1 -> sim_out/1
  out_reg/1 -> sim_out_reg_sim_delay/1, assert_reg/1
  assert_reg/1 -> reint1/1
  reint1/1 -> io_delay/1
